simulink model "drive_esc"  (R2026b)
settings: Solver=VariableStepAuto
undefined symbols (not defined in the file or in its folder): DiscIntNeverNeededParam, P
libraries: simulink x14, mcbpccprotrelaylib x10, sl_discontinuities x2, mcbpccswwdtimerlib x1, slpidlib x1
settings Model: Creator=aomar  LastModifiedBy=aomar

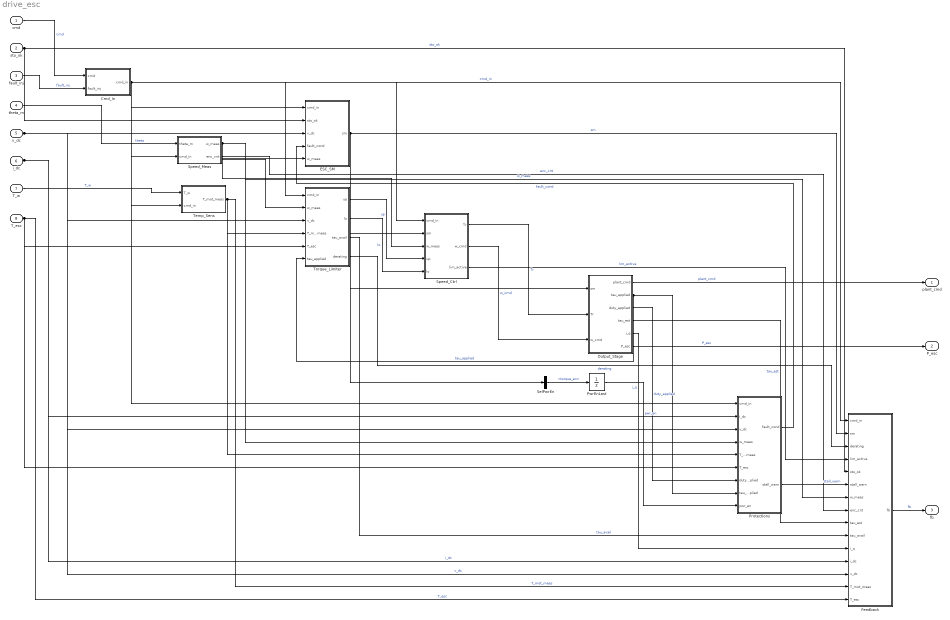
== system drive_esc ==
  cmd : Inport  OutDataTypeStr=Bus: Bus_DriveSideCmd  SampleTime=P.drive.Ts_esc
  sto_ok : Inport  Port=2  OutDataTypeStr=boolean  SampleTime=P.drive.Ts_esc
  fault_inj : Inport  Port=3  OutDataTypeStr=Bus: Bus_DriveSideFaultInj  SampleTime=P.drive.Ts_esc
  theta_m : Inport  Port=4  OutDataTypeStr=double  SampleTime=P.drive.Ts_esc
  v_dc : Inport  Port=5  OutDataTypeStr=double  SampleTime=P.drive.Ts_esc
  i_dc : Inport  Port=6  OutDataTypeStr=double  SampleTime=P.drive.Ts_esc
  T_w : Inport  Port=7  OutDataTypeStr=double  SampleTime=P.drive.Ts_esc
  T_esc : Inport  Port=8  OutDataTypeStr=double  SampleTime=P.drive.Ts_esc
  Cmd_In : Subsystem
  ESC_SM : Subsystem
  Feedback : Subsystem
  Output_Stage : Subsystem
  Protections : Subsystem
  PwrEnLast : UnitDelay  InitialCondition=false  SampleTime=P.drive.Ts_esc
  SelPwrEn : BusSelector  OutputSignals=torque_en
  Speed_Ctrl : Subsystem
  Speed_Meas : Subsystem
  Temp_Sens : Subsystem
  Torque_Limiter : Subsystem
  plant_cmd : Outport  OutDataTypeStr=double
  P_esc : Outport  Port=2  OutDataTypeStr=double
  fb : Outport  Port=3  OutDataTypeStr=Bus: Bus_DriveSideFb
  wires:
  cmd/1 -> Cmd_In/1(cmd)  "cmd"
  sto_ok/1 -> Feedback/5(sto_ok), ESC_SM/2(sto_ok)  "sto_ok"
  fault_inj/1 -> Cmd_In/2(fault_inj)  "fault_inj"
  theta_m/1 -> Speed_Meas/1(theta_m)  "theta"
  T_w/1 -> Temp_Sens/1(T_w)  "T_w"
  Cmd_In/1(cmd_in) -> Feedback/1(cmd_in), Protections/1(cmd_in), Speed_Ctrl/1(cmd_in), Temp_Sens/2(cmd_in), Torque_Limiter/1(cmd_in), Speed_Meas/2(cmd_in), ESC_SM/1(cmd_in)  "cmd_in"
  Speed_Meas/1(w_meas) -> Feedback/7(w_meas), Protections/4(w_meas), Speed_Ctrl/3(w_meas), Torque_Limiter/2(w_meas), ESC_SM/5(w_meas)  "w_meas"
  Speed_Meas/2(enc_cnt) -> Feedback/8(enc_cnt)  "enc_cnt"
  Temp_Sens/1(T_mot_meas) -> Feedback/14(T_mot_meas), Protections/5(T_mot_meas), Torque_Limiter/4(T_mot_meas)  "T_mot_meas"
  ESC_SM/1(sm) -> Feedback/2(sm), SelPwrEn/1, Output_Stage/1(sm), Speed_Ctrl/2(sm)  "sm"
  Torque_Limiter/1(up) -> Speed_Ctrl/4(up)  "up"
  Torque_Limiter/2(lo) -> Speed_Ctrl/5(lo)  "lo"
  Torque_Limiter/3(tau_avail) -> Feedback/10(tau_avail)  "tau_avail"
  Torque_Limiter/4(derating) -> Feedback/3(derating)  "derating"
  Speed_Ctrl/1(Tr) -> Output_Stage/2(Tr)  "Tr"
  Speed_Ctrl/2(w_cmd) -> Output_Stage/3(w_cmd)  "w_cmd"
  Speed_Ctrl/3(lim_active) -> Feedback/4(lim_active)  "lim_active"
  SelPwrEn/1 -> PwrEnLast/1  "<torque_en>"
  PwrEnLast/1 -> Protections/9(pwr_en)  "pwr_en"
  Output_Stage/1(plant_cmd) -> plant_cmd/1  "plant_cmd"
  Output_Stage/2(tau_applied) -> Protections/8(tau_applied), Torque_Limiter/6(tau_applied)  "tau_applied"
  Output_Stage/3(duty_applied) -> Protections/7(duty_applied)  "duty_applied"
  Output_Stage/4(tau_est) -> Feedback/9(tau_est)  "tau_est"
  Output_Stage/5(i_q) -> Feedback/11(i_q)  "i_q"
  Output_Stage/6(P_esc) -> P_esc/1  "P_esc"
  Protections/1(fault_cond) -> ESC_SM/4(fault_cond)  "fault_cond"
  Protections/2(stall_warn) -> Feedback/6(stall_warn)  "stall_warn"
  Feedback/1(fb) -> fb/1  "fb"
  v_dc/1 -> Feedback/13(v_dc), Protections/3(v_dc), Torque_Limiter/3(v_dc), ESC_SM/3(v_dc)  "v_dc"
  i_dc/1 -> Feedback/12(i_dc), Protections/2(i_dc)  "i_dc"
  T_esc/1 -> Feedback/15(T_esc), Protections/6(T_esc), Torque_Limiter/5(T_esc)  "T_esc"

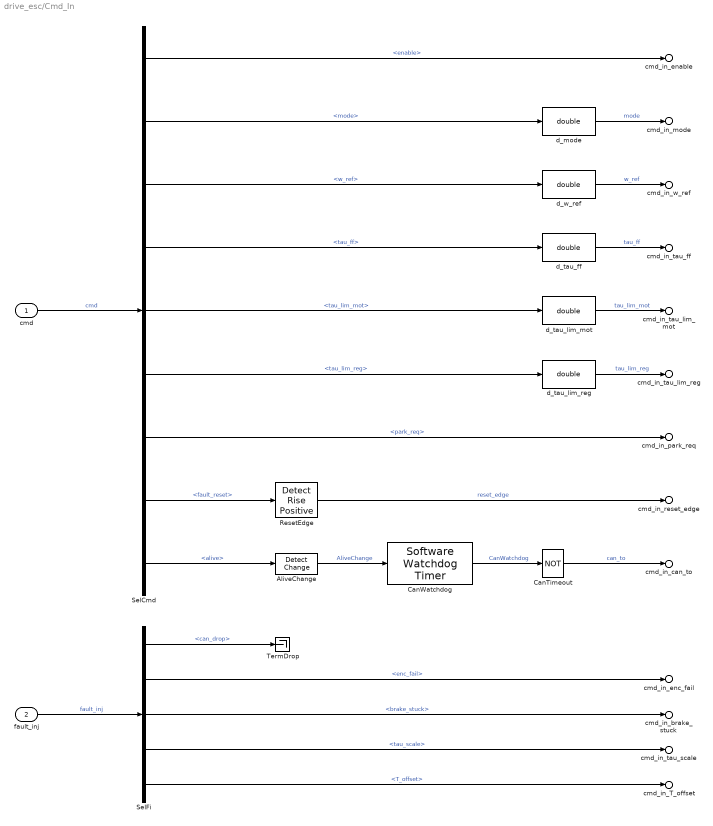
== system drive_esc/Cmd_In ==
  cmd : Inport
  fault_inj : Inport  Port=2
  AliveChange : simulink/Logic and Bit Operations/Detect Change  vinit=0  OutDataTypeStr=boolean
  CanTimeout : Logic  Operator=NOT  Inputs=1  AllPortsSameDT=off  OutDataTypeStr=boolean
  CanWatchdog : mcbpccswwdtimerlib/Software Watchdog Timer  maxCountInput=Specify via dialog  maxCount=P.drive.esc.n_can_to  datatype=uint8
      settings: LibrarySourceBlock=mcblib/Protection and Diagnostics/Software Watchdog Timer
  ResetEdge : simulink/Logic and Bit Operations/Detect Rise Positive  vinit=0  OutDataTypeStr=boolean
  SelCmd : BusSelector  OutputSignals=enable,mode,w_ref,tau_ff,tau_lim_mot,tau_lim_reg,park_req,fault_reset,alive
  SelFi : BusSelector  OutputSignals=can_drop,enc_fail,brake_stuck,tau_scale,T_offset
  TermDrop : Terminator
  d_mode : DataTypeConversion  OutDataTypeStr=double  RndMeth=Nearest
  d_tau_ff : DataTypeConversion  OutDataTypeStr=double  RndMeth=Nearest
  d_tau_lim_mot : DataTypeConversion  OutDataTypeStr=double  RndMeth=Nearest
  d_tau_lim_reg : DataTypeConversion  OutDataTypeStr=double  RndMeth=Nearest
  d_w_ref : DataTypeConversion  OutDataTypeStr=double  RndMeth=Nearest
  cmd_in_enable : Outport  PortName=cmd_in  Element=enable
  cmd_in_mode : Outport  PortName=cmd_in  Element=mode
  cmd_in_w_ref : Outport  PortName=cmd_in  Element=w_ref
  cmd_in_tau_ff : Outport  PortName=cmd_in  Element=tau_ff
  cmd_in_tau_lim_mot : Outport  PortName=cmd_in  Element=tau_lim_mot
  cmd_in_tau_lim_reg : Outport  PortName=cmd_in  Element=tau_lim_reg
  cmd_in_park_req : Outport  PortName=cmd_in  Element=park_req
  cmd_in_reset_edge : Outport  PortName=cmd_in  Element=reset_edge
  cmd_in_can_to : Outport  PortName=cmd_in  Element=can_to
  cmd_in_enc_fail : Outport  PortName=cmd_in  Element=enc_fail
  cmd_in_brake_stuck : Outport  PortName=cmd_in  Element=brake_stuck
  cmd_in_tau_scale : Outport  PortName=cmd_in  Element=tau_scale
  cmd_in_T_offset : Outport  PortName=cmd_in  Element=T_offset
  wires:
  cmd/1 -> SelCmd/1  "cmd"
  fault_inj/1 -> SelFi/1  "fault_inj"
  SelCmd/1 -> cmd_in_enable/1  "<enable>"
  SelCmd/2 -> d_mode/1  "<mode>"
  SelCmd/3 -> d_w_ref/1  "<w_ref>"
  SelCmd/4 -> d_tau_ff/1  "<tau_ff>"
  SelCmd/5 -> d_tau_lim_mot/1  "<tau_lim_mot>"
  SelCmd/6 -> d_tau_lim_reg/1  "<tau_lim_reg>"
  SelCmd/7 -> cmd_in_park_req/1  "<park_req>"
  SelCmd/8 -> ResetEdge/1  "<fault_reset>"
  SelCmd/9 -> AliveChange/1  "<alive>"
  SelFi/1 -> TermDrop/1  "<can_drop>"
  SelFi/2 -> cmd_in_enc_fail/1  "<enc_fail>"
  SelFi/3 -> cmd_in_brake_stuck/1  "<brake_stuck>"
  SelFi/4 -> cmd_in_tau_scale/1  "<tau_scale>"
  SelFi/5 -> cmd_in_T_offset/1  "<T_offset>"
  ResetEdge/1 -> cmd_in_reset_edge/1  "reset_edge"
  AliveChange/1 -> CanWatchdog/1  "AliveChange"
  CanWatchdog/1 -> CanTimeout/1  "CanWatchdog"
  CanTimeout/1 -> cmd_in_can_to/1  "can_to"
  d_mode/1 -> cmd_in_mode/1  "mode"
  d_w_ref/1 -> cmd_in_w_ref/1  "w_ref"
  d_tau_ff/1 -> cmd_in_tau_ff/1  "tau_ff"
  d_tau_lim_mot/1 -> cmd_in_tau_lim_mot/1  "tau_lim_mot"
  d_tau_lim_reg/1 -> cmd_in_tau_lim_reg/1  "tau_lim_reg"

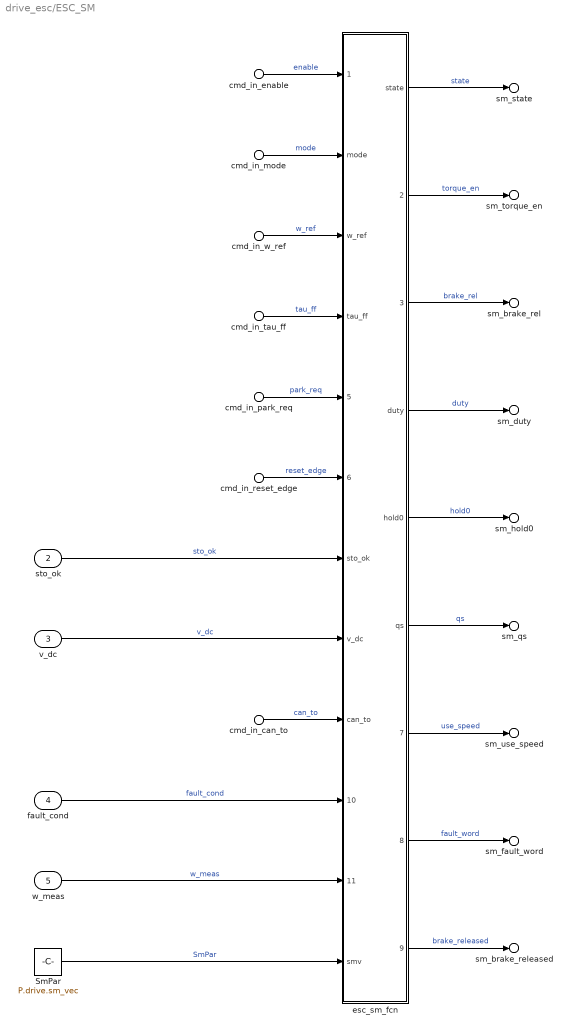
== system drive_esc/ESC_SM ==
  cmd_in_enable : Inport  PortName=cmd_in  Element=enable
  cmd_in_mode : Inport  PortName=cmd_in  Element=mode
  cmd_in_w_ref : Inport  PortName=cmd_in  Element=w_ref
  cmd_in_tau_ff : Inport  PortName=cmd_in  Element=tau_ff
  cmd_in_park_req : Inport  PortName=cmd_in  Element=park_req
  cmd_in_reset_edge : Inport  PortName=cmd_in  Element=reset_edge
  cmd_in_can_to : Inport  PortName=cmd_in  Element=can_to
  sto_ok : Inport  Port=2
  v_dc : Inport  Port=3
  fault_cond : Inport  Port=4
  w_meas : Inport  Port=5
  SmPar : Constant  Value=P.drive.sm_vec  OutDataTypeStr=double
  esc_sm_fcn : MATLAB Function  TreatAsAtomicUnit=on
  sm_state : Outport  PortName=sm  Element=state
  sm_torque_en : Outport  PortName=sm  Element=torque_en
  sm_brake_rel : Outport  PortName=sm  Element=brake_rel
  sm_duty : Outport  PortName=sm  Element=duty
  sm_hold0 : Outport  PortName=sm  Element=hold0
  sm_qs : Outport  PortName=sm  Element=qs
  sm_use_speed : Outport  PortName=sm  Element=use_speed
  sm_fault_word : Outport  PortName=sm  Element=fault_word
  sm_brake_released : Outport  PortName=sm  Element=brake_released
  wires:
  sto_ok/1 -> esc_sm_fcn/7(sto_ok)  "sto_ok"
  v_dc/1 -> esc_sm_fcn/8(v_dc)  "v_dc"
  fault_cond/1 -> esc_sm_fcn/10(fault_cond)  "fault_cond"
  w_meas/1 -> esc_sm_fcn/11(w_meas)  "w_meas"
  SmPar/1 -> esc_sm_fcn/12(smv)  "SmPar"
  cmd_in_enable/1 -> esc_sm_fcn/1(enable)  "enable"
  cmd_in_mode/1 -> esc_sm_fcn/2(mode)  "mode"
  cmd_in_w_ref/1 -> esc_sm_fcn/3(w_ref)  "w_ref"
  cmd_in_tau_ff/1 -> esc_sm_fcn/4(tau_ff)  "tau_ff"
  cmd_in_park_req/1 -> esc_sm_fcn/5(park_req)  "park_req"
  cmd_in_reset_edge/1 -> esc_sm_fcn/6(reset_edge)  "reset_edge"
  cmd_in_can_to/1 -> esc_sm_fcn/9(can_to)  "can_to"
  esc_sm_fcn/1(state) -> sm_state/1  "state"
  esc_sm_fcn/2(torque_en) -> sm_torque_en/1  "torque_en"
  esc_sm_fcn/3(brake_rel) -> sm_brake_rel/1  "brake_rel"
  esc_sm_fcn/4(duty) -> sm_duty/1  "duty"
  esc_sm_fcn/5(hold0) -> sm_hold0/1  "hold0"
  esc_sm_fcn/6(qs) -> sm_qs/1  "qs"
  esc_sm_fcn/7(use_speed) -> sm_use_speed/1  "use_speed"
  esc_sm_fcn/8(fault_word) -> sm_fault_word/1  "fault_word"
  esc_sm_fcn/9(brake_released) -> sm_brake_released/1  "brake_released"

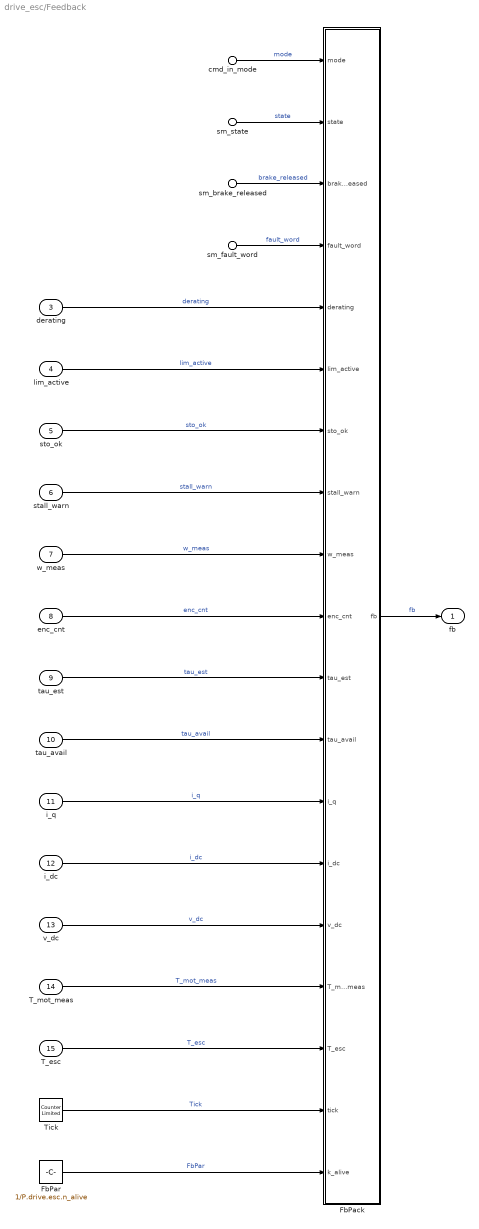
== system drive_esc/Feedback ==
  cmd_in_mode : Inport  PortName=cmd_in  Element=mode
  sm_state : Inport  Port=2  PortName=sm  Element=state
  sm_brake_released : Inport  Port=2  PortName=sm  Element=brake_released
  sm_fault_word : Inport  Port=2  PortName=sm  Element=fault_word
  derating : Inport  Port=3
  lim_active : Inport  Port=4
  sto_ok : Inport  Port=5
  stall_warn : Inport  Port=6
  w_meas : Inport  Port=7
  enc_cnt : Inport  Port=8
  tau_est : Inport  Port=9
  tau_avail : Inport  Port=10
  i_q : Inport  Port=11
  i_dc : Inport  Port=12
  v_dc : Inport  Port=13
  T_mot_meas : Inport  Port=14
  T_esc : Inport  Port=15
  FbPack : MATLAB Function  TreatAsAtomicUnit=on
  FbPar : Constant  Value=1/P.drive.esc.n_alive  OutDataTypeStr=double
  Tick : simulink/Sources/Counter Limited  uplimit=256*P.drive.esc.n_alive - 1  tsamp=P.drive.Ts_esc
  fb : Outport
  wires:
  derating/1 -> FbPack/5(derating)  "derating"
  lim_active/1 -> FbPack/6(lim_active)  "lim_active"
  sto_ok/1 -> FbPack/7(sto_ok)  "sto_ok"
  stall_warn/1 -> FbPack/8(stall_warn)  "stall_warn"
  w_meas/1 -> FbPack/9(w_meas)  "w_meas"
  enc_cnt/1 -> FbPack/10(enc_cnt)  "enc_cnt"
  tau_est/1 -> FbPack/11(tau_est)  "tau_est"
  tau_avail/1 -> FbPack/12(tau_avail)  "tau_avail"
  i_q/1 -> FbPack/13(i_q)  "i_q"
  i_dc/1 -> FbPack/14(i_dc)  "i_dc"
  v_dc/1 -> FbPack/15(v_dc)  "v_dc"
  T_mot_meas/1 -> FbPack/16(T_mot_meas)  "T_mot_meas"
  T_esc/1 -> FbPack/17(T_esc)  "T_esc"
  Tick/1 -> FbPack/18(tick)  "Tick"
  FbPar/1 -> FbPack/19(k_alive)  "FbPar"
  cmd_in_mode/1 -> FbPack/1(mode)  "mode"
  sm_state/1 -> FbPack/2(state)  "state"
  sm_brake_released/1 -> FbPack/3(brake_released)  "brake_released"
  sm_fault_word/1 -> FbPack/4(fault_word)  "fault_word"
  FbPack/1(fb) -> fb/1  "fb"

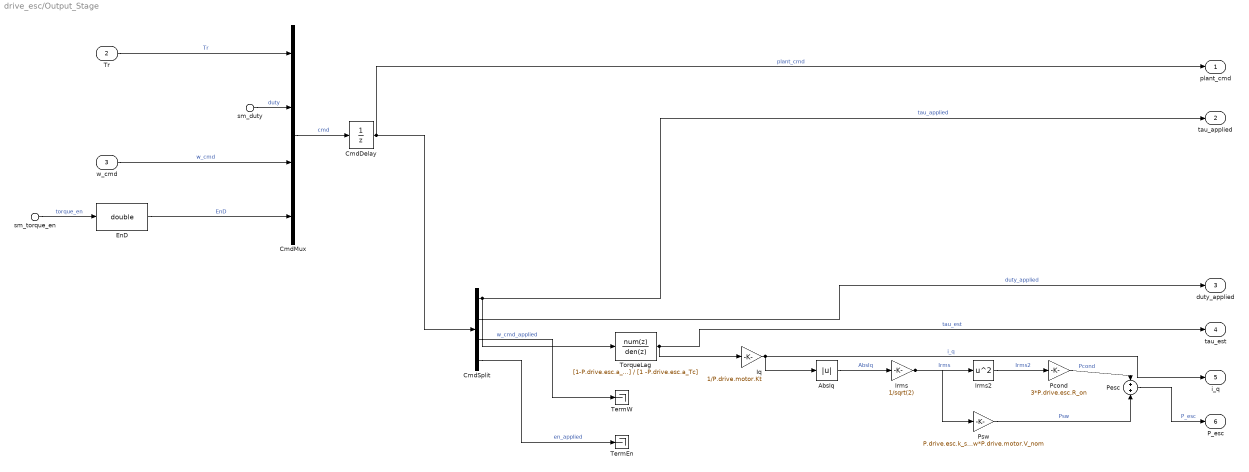
== system drive_esc/Output_Stage ==
  sm_duty : Inport  PortName=sm  Element=duty
  sm_torque_en : Inport  PortName=sm  Element=torque_en
  Tr : Inport  Port=2
  w_cmd : Inport  Port=3
  AbsIq : Abs  SaturateOnIntegerOverflow=off
  CmdDelay : UnitDelay  InitialCondition=zeros(4,1)  SampleTime=P.drive.Ts_esc
  CmdMux : Mux
  CmdSplit : Demux
  EnD : DataTypeConversion  OutDataTypeStr=double  RndMeth=Nearest
  Iq : Gain  Gain=1/P.drive.motor.Kt
  Irms : Gain  Gain=1/sqrt(2)
  Irms2 : Math  Operator=square
  Pcond : Gain  Gain=3*P.drive.esc.R_on
  Pesc : Sum
  Psw : Gain  Gain=P.drive.esc.k_sw*P.drive.motor.V_nom
  TermEn : Terminator
  TermW : Terminator
  TorqueLag : DiscreteTransferFcn  Numerator=[1-P.drive.esc.a_Tc]  Denominator=[1 -P.drive.esc.a_Tc]  SampleTime=P.drive.Ts_esc
  plant_cmd : Outport
  tau_applied : Outport  Port=2
  duty_applied : Outport  Port=3
  tau_est : Outport  Port=4
  i_q : Outport  Port=5
  P_esc : Outport  Port=6
  wires:
  sm_torque_en/1 -> EnD/1  "torque_en"
  Tr/1 -> CmdMux/1  "Tr"
  w_cmd/1 -> CmdMux/3  "w_cmd"
  EnD/1 -> CmdMux/4  "EnD"
  sm_duty/1 -> CmdMux/2  "duty"
  CmdMux/1 -> CmdDelay/1  "cmd"
  CmdDelay/1 -> CmdSplit/1, plant_cmd/1  "plant_cmd"
  CmdSplit/1 -> tau_applied/1, TorqueLag/1  "tau_applied"
  CmdSplit/2 -> duty_applied/1  "duty_applied"
  CmdSplit/3 -> TermW/1  "w_cmd_applied"
  CmdSplit/4 -> TermEn/1  "en_applied"
  TorqueLag/1 -> tau_est/1, Iq/1  "tau_est"
  Iq/1 -> i_q/1, AbsIq/1  "i_q"
  AbsIq/1 -> Irms/1  "AbsIq"
  Irms/1 -> Psw/1, Irms2/1  "Irms"
  Irms2/1 -> Pcond/1  "Irms2"
  Psw/1 -> Pesc/2  "Psw"
  Pcond/1 -> Pesc/1  "Pcond"
  Pesc/1 -> P_esc/1  "P_esc"

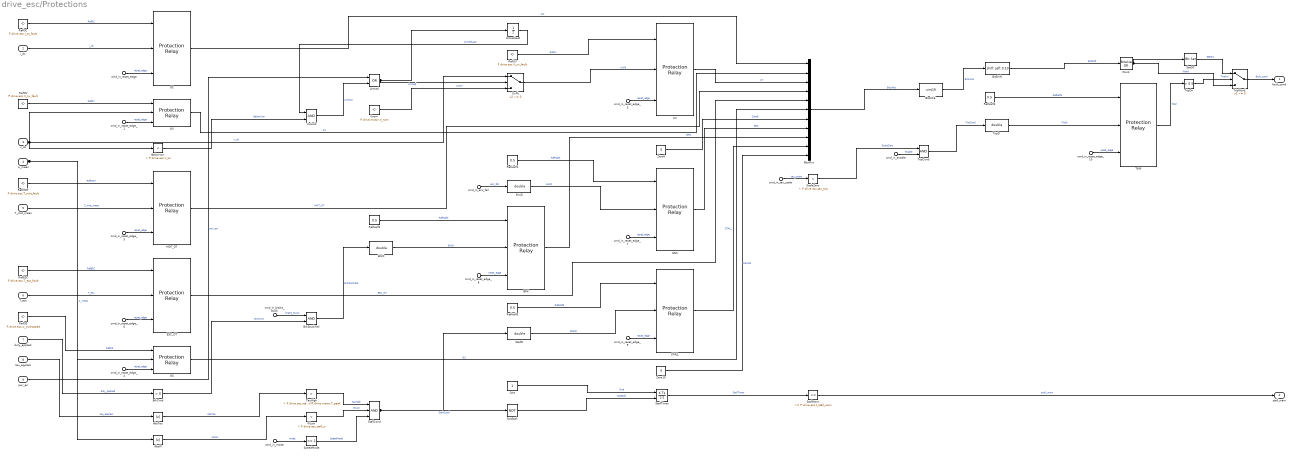
== system drive_esc/Protections ==
  cmd_in_enc_fail : Inport  PortName=cmd_in  Element=enc_fail
  cmd_in_brake_stuck : Inport  PortName=cmd_in  Element=brake_stuck
  cmd_in_mode : Inport  PortName=cmd_in  Element=mode
  cmd_in_tau_scale : Inport  PortName=cmd_in  Element=tau_scale
  cmd_in_enable : Inport  PortName=cmd_in  Element=enable
  cmd_in_reset_edge : Inport  PortName=cmd_in  Element=reset_edge
  cmd_in_reset_edge_{2..10} (9 alike) : Inport  PortName=cmd_in  Element=reset_edge
  i_dc : Inport  Port=2
  v_dc : Inport  Port=3
  w_meas : Inport  Port=4
  T_mot_meas : Inport  Port=5
  T_esc : Inport  Port=6
  duty_applied : Inport  Port=7
  tau_applied : Inport  Port=8
  pwr_en : Inport  Port=9
  AbsTau : Abs  SaturateOnIntegerOverflow=off
  AbsW : Abs  SaturateOnIntegerOverflow=off
  Armed : Logic  Operator=OR  AllPortsSameDT=off  OutDataTypeStr=boolean
  ArmedLast : UnitDelay  InitialCondition=false  SampleTime=P.drive.Ts_esc
  BRK : mcbpccprotrelaylib/Protection Relay  Protection=Overvoltage  CountMaxInputType=Specify via dialog  CountMax=P.drive.esc.n_brake  SamplesForDebounce=0
      settings: LibrarySourceBlock=mcblib/Protection and Diagnostics/Protection Relay
  BelowVon : simulink/Logic and Bit Operations/Compare To Constant  relop=<  const=P.drive.esc.V_on  OutDataTypeStr=boolean
  BitShift : ArithShift  BitShiftNumber=0:10  BitShiftDirection=Left
  BitsMux : Mux  Inputs=11
  BitsU16 : DataTypeConversion  OutDataTypeStr=uint16  RndMeth=Nearest
  BrkCmd : simulink/Logic and Bit Operations/Compare To Constant  relop=>  const=0  OutDataTypeStr=boolean
  BrkD : DataTypeConversion  OutDataTypeStr=double  RndMeth=Nearest
  BrkStuckRel : Logic  AllPortsSameDT=off  OutDataTypeStr=boolean
  ENC : mcbpccprotrelaylib/Protection Relay  Protection=Overvoltage  CountMaxInputType=Specify via dialog  CountMax=P.drive.esc.n_enc  SamplesForDebounce=0
      settings: LibrarySourceBlock=mcblib/Protection and Diagnostics/Protection Relay
  ESC_OT : mcbpccprotrelaylib/Protection Relay  Protection=Overvoltage  CountMaxInputType=Specify via dialog  CountMax=P.drive.esc.n_ot  SamplesForDebounce=0
      settings: LibrarySourceBlock=mcblib/Protection and Diagnostics/Protection Relay
  EncD : DataTypeConversion  OutDataTypeStr=double  RndMeth=Nearest
  MOT_OT : mcbpccprotrelaylib/Protection Relay  Protection=Overvoltage  CountMaxInputType=Specify via dialog  CountMax=P.drive.esc.n_ot  SamplesForDebounce=0
      settings: LibrarySourceBlock=mcblib/Protection and Diagnostics/Protection Relay
  NotStall : Logic  Operator=NOT  Inputs=1  AllPortsSameDT=off  OutDataTypeStr=boolean
  OC : mcbpccprotrelaylib/Protection Relay  Protection=Overcurrent  CountMaxInputType=Specify via dialog  CountMax=P.drive.esc.n_oc  SamplesForDebounce=0
      settings: LibrarySourceBlock=mcblib/Protection and Diagnostics/Protection Relay
  OS : mcbpccprotrelaylib/Protection Relay  Protection=Overspeed  CountMaxInputType=Specify via dialog  CountMax=P.drive.esc.n_os  SamplesForDebounce=0
      settings: LibrarySourceBlock=mcblib/Protection and Diagnostics/Protection Relay
  OV : mcbpccprotrelaylib/Protection Relay  Protection=Overvoltage  CountMaxInputType=Specify via dialog  CountMax=P.drive.esc.n_ov  SamplesForDebounce=0
      settings: LibrarySourceBlock=mcblib/Protection and Diagnostics/Protection Relay
  One : Constant
  RefESC : Constant  Value=P.drive.esc.T_esc_fault
  RefHalf{1..4} (4 alike) : Constant  Value=0.5
  RefMOT : Constant  Value=P.drive.esc.T_mot_fault
  RefOC : Constant  Value=P.drive.esc.I_oc_fault
  RefOS : Constant  Value=P.drive.esc.w_overspeed
  RefOV : Constant  Value=P.drive.esc.V_ov_fault
  RefUV : Constant  Value=P.drive.esc.V_uv_fault
  STALL : mcbpccprotrelaylib/Protection Relay  Protection=Overvoltage  CountMaxInputType=Specify via dialog  CountMax=P.drive.esc.n_stall  SamplesForDebounce=0
      settings: LibrarySourceBlock=mcblib/Protection and Diagnostics/Protection Relay
  ScaleZero : simulink/Logic and Bit Operations/Compare To Constant  relop=<  const=P.drive.esc.tau_trip  OutDataTypeStr=boolean
  SetOC : simulink/Logic and Bit Operations/Bit Set  iBit=0
  SpeedMode : simulink/Logic and Bit Operations/Compare To Constant  relop===  const=1  OutDataTypeStr=boolean
  StallCond : Logic  Inputs=3  AllPortsSameDT=off  OutDataTypeStr=boolean
  StallD : DataTypeConversion  OutDataTypeStr=double  RndMeth=Nearest
  StallTimer : DiscreteIntegrator  ExternalReset=level  SampleTime=P.drive.Ts_esc  ICPrevOutput=DiscIntNeverNeededParam  ICPrevScaledInput=DiscIntNeverNeededParam
  StallWarn : simulink/Logic and Bit Operations/Compare To Constant  relop=>=  const=P.drive.esc.t_stall_warn  OutDataTypeStr=boolean
  TRIP : mcbpccprotrelaylib/Protection Relay  Protection=Overvoltage  CountMaxInputType=Specify via dialog  CountMax=1  SamplesForDebounce=0
      settings: LibrarySourceBlock=mcblib/Protection and Diagnostics/Protection Relay
  TauHigh : simulink/Logic and Bit Operations/Compare To Constant  relop=>  const=P.drive.esc.stall_tau_frac*P.drive.motor.T_peak  OutDataTypeStr=boolean
  TripCond : Logic  AllPortsSameDT=off  OutDataTypeStr=boolean
  TripD : DataTypeConversion  OutDataTypeStr=double  RndMeth=Nearest
  TripOn : simulink/Logic and Bit Operations/Compare To Constant  relop=>  const=0.5  OutDataTypeStr=boolean
  TripWord : Switch  Criteria=u2 ~= 0  SaturateOnIntegerOverflow=off  InputSameDT=off
  UV : mcbpccprotrelaylib/Protection Relay  Protection=Undervoltage  CountMaxInputType=Specify via dialog  CountMax=P.drive.esc.n_uv  SamplesForDebounce=0
      settings: LibrarySourceBlock=mcblib/Protection and Diagnostics/Protection Relay
  UvFb : Switch  Criteria=u2 ~= 0  SaturateOnIntegerOverflow=off  InputSameDT=off
  UvHold : Logic  AllPortsSameDT=off  OutDataTypeStr=boolean
  Vnom : Constant  Value=P.drive.motor.V_nom
  WLow : simulink/Logic and Bit Operations/Compare To Constant  relop=<  const=P.drive.esc.stall_w  OutDataTypeStr=boolean
  Word : simulink/Logic and Bit Operations/Bitwise Operator  logicop=OR  UseBitMask=off  BitMask=bin2dec('11011001')  BitMaskRealWorld=Stored Integer
  Zero10 : Constant  Value=0
  Zero6 : Constant  Value=0
  fault_cond : Outport
  stall_warn : Outport  Port=2
  wires:
  RefOC/1 -> OC/1  "RefOC"
  i_dc/1 -> OC/2  "i_dc"
  RefOV/1 -> OV/1  "RefOV"
  v_dc/1 -> UvFb/1, OV/2, BelowVon/1  "v_dc"
  w_meas/1 -> AbsW/1, OS/2  "w_meas"
  RefMOT/1 -> MOT_OT/1  "RefMOT"
  T_mot_meas/1 -> MOT_OT/2  "T_mot_meas"
  RefESC/1 -> ESC_OT/1  "RefESC"
  T_esc/1 -> ESC_OT/2  "T_esc"
  RefOS/1 -> OS/1  "RefOS"
  duty_applied/1 -> BrkCmd/1  "duty_applied"
  tau_applied/1 -> AbsTau/1  "tau_applied"
  pwr_en/1 -> Armed/1  "pwr_en"
  cmd_in_reset_edge/1 -> OC/3  "reset_edge"
  cmd_in_reset_edge_2/1 -> OV/3  "reset_edge"
  cmd_in_reset_edge_5/1 -> MOT_OT/3  "reset_edge"
  cmd_in_reset_edge_6/1 -> ESC_OT/3  "reset_edge"
  cmd_in_reset_edge_4/1 -> OS/3  "reset_edge"
  BelowVon/1 -> UvHold/2  "BelowVon"
  BrkCmd/1 -> BrkStuckRel/2  "BrkCmd"
  AbsTau/1 -> TauHigh/1  "AbsTau"
  AbsW/1 -> WLow/1  "AbsW"
  OC/1 -> BitsMux/1  "OC"
  OV/1 -> BitsMux/2  "OV"
  MOT_OT/1 -> BitsMux/4  "MOT_OT"
  ESC_OT/1 -> BitsMux/5  "ESC_OT"
  OS/1 -> BitsMux/6  "OS"
  cmd_in_brake_stuck/1 -> BrkStuckRel/1  "brake_stuck"
  cmd_in_mode/1 -> SpeedMode/1  "mode"
  UvHold/1 -> Armed/2  "UvHold"
  BrkStuckRel/1 -> BrkD/1  "BrkStuckRel"
  TauHigh/1 -> StallCond/1  "TauHigh"
  WLow/1 -> StallCond/2  "WLow"
  SpeedMode/1 -> StallCond/3  "SpeedMode"
  Armed/1 -> ArmedLast/1, UvFb/2  "Armed"
  Vnom/1 -> UvFb/3  "Vnom"
  RefHalf2/1 -> BRK/1  "RefHalf2"
  StallCond/1 -> StallD/1, NotStall/1  "StallCond"
  BrkD/1 -> BRK/2  "BrkD"
  cmd_in_enc_fail/1 -> EncD/1  "enc_fail"
  cmd_in_reset_edge_8/1 -> BRK/3  "reset_edge"
  RefUV/1 -> UV/1  "RefUV"
  RefHalf1/1 -> ENC/1  "RefHalf1"
  RefHalf3/1 -> STALL/1  "RefHalf3"
  One/1 -> StallTimer/1  "One"
  NotStall/1 -> StallTimer/2  "NotStall"
  ArmedLast/1 -> UvHold/1  "ArmedLast"
  UvFb/1 -> UV/2  "UvFb"
  EncD/1 -> ENC/2  "EncD"
  StallD/1 -> STALL/2  "StallD"
  BRK/1 -> BitsMux/9  "BRK"
  cmd_in_reset_edge_3/1 -> UV/3  "reset_edge"
  cmd_in_reset_edge_7/1 -> ENC/3  "reset_edge"
  cmd_in_reset_edge_9/1 -> STALL/3  "reset_edge"
  Zero6/1 -> BitsMux/7  "Zero6"
  Zero10/1 -> BitsMux/11  "Zero10"
  StallTimer/1 -> StallWarn/1  "StallTimer"
  UV/1 -> BitsMux/3  "UV"
  ENC/1 -> BitsMux/8  "ENC"
  STALL/1 -> BitsMux/10  "STALL"
  cmd_in_tau_scale/1 -> ScaleZero/1  "tau_scale"
  BitsMux/1 -> BitsU16/1  "BitsMux"
  ScaleZero/1 -> TripCond/1  "ScaleZero"
  StallWarn/1 -> stall_warn/1  "stall_warn"
  cmd_in_enable/1 -> TripCond/2  "enable"
  TripCond/1 -> TripD/1  "TripCond"
  BitsU16/1 -> BitShift/1  "BitsU16"
  RefHalf4/1 -> TRIP/1  "RefHalf4"
  TripD/1 -> TRIP/2  "TripD"
  BitShift/1 -> Word/1  "BitShift"
  cmd_in_reset_edge_10/1 -> TRIP/3  "reset_edge"
  Word/1 -> TripWord/3, SetOC/1  "Word"
  TRIP/1 -> TripOn/1  "TRIP"
  TripOn/1 -> TripWord/2  "TripOn"
  SetOC/1 -> TripWord/1  "SetOC"
  TripWord/1 -> fault_cond/1  "fault_cond"

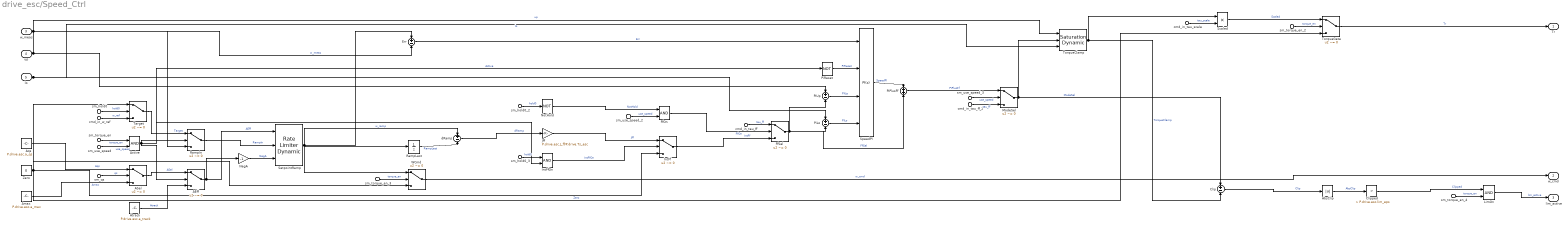
== system drive_esc/Speed_Ctrl ==
  cmd_in_w_ref : Inport  PortName=cmd_in  Element=w_ref
  cmd_in_tau_ff : Inport  PortName=cmd_in  Element=tau_ff
  cmd_in_tau_ff_2 : Inport  PortName=cmd_in  Element=tau_ff
  cmd_in_tau_scale : Inport  PortName=cmd_in  Element=tau_scale
  sm_hold0 : Inport  Port=2  PortName=sm  Element=hold0
  sm_hold0_2 : Inport  Port=2  PortName=sm  Element=hold0
  sm_hold0_3 : Inport  Port=2  PortName=sm  Element=hold0
  sm_torque_en : Inport  Port=2  PortName=sm  Element=torque_en
  sm_torque_en_2 : Inport  Port=2  PortName=sm  Element=torque_en
  sm_torque_en_3 : Inport  Port=2  PortName=sm  Element=torque_en
  sm_torque_en_4 : Inport  Port=2  PortName=sm  Element=torque_en
  sm_use_speed : Inport  Port=2  PortName=sm  Element=use_speed
  sm_use_speed_2 : Inport  Port=2  PortName=sm  Element=use_speed
  sm_use_speed_3 : Inport  Port=2  PortName=sm  Element=use_speed
  sm_qs : Inport  Port=2  PortName=sm  Element=qs
  w_meas : Inport  Port=3
  up : Inport  Port=4
  lo : Inport  Port=5
  AEff : Switch  Criteria=u2 ~= 0  SaturateOnIntegerOverflow=off  InputSameDT=off
  ASel : Switch  Criteria=u2 ~= 0  SaturateOnIntegerOverflow=off  InputSameDT=off
  AbsClip : Abs  SaturateOnIntegerOverflow=off
  Active : Logic  AllPortsSameDT=off  OutDataTypeStr=boolean
  Amax : Constant  Value=P.drive.esc.a_max
  Aqs : Constant  Value=P.drive.esc.a_qs
  Atrack : Constant  Value=P.drive.esc.a_track
  Clip : Sum  Inputs=+-
  Clipped : simulink/Logic and Bit Operations/Compare To Constant  relop=>  const=P.drive.esc.lim_eps  OutDataTypeStr=boolean
  Err : Sum  Inputs=+-
  FfOn : Logic  AllPortsSameDT=off  OutDataTypeStr=boolean
  FfSel : Switch  Criteria=u2 ~= 0  SaturateOnIntegerOverflow=off  InputSameDT=off
  IntFf : Switch  Criteria=u2 ~= 0  SaturateOnIntegerOverflow=off  InputSameDT=off
  IntFfOn : Logic  AllPortsSameDT=off  OutDataTypeStr=boolean
  Jff : Gain  Gain=P.drive.esc.J_ff/P.drive.Ts_esc
  LimOn : Logic  AllPortsSameDT=off  OutDataTypeStr=boolean
  ModeSel : Switch  Criteria=u2 ~= 0  SaturateOnIntegerOverflow=off  InputSameDT=off
  NegA : Gain  Gain=-1
  NotHold : Logic  Operator=NOT  Inputs=1  AllPortsSameDT=off  OutDataTypeStr=boolean
  PiLo : Sum  Inputs=+-
  PiPlusFf : Sum
  PiReset : Logic  Operator=NOT  Inputs=1  AllPortsSameDT=off  OutDataTypeStr=boolean
  PiUp : Sum  Inputs=+-
  RampIn : Switch  Criteria=u2 ~= 0  SaturateOnIntegerOverflow=off  InputSameDT=off
  RampLast : UnitDelay  SampleTime=P.drive.Ts_esc
  Scaled : Product  Inputs=**
  SetpointRamp : sl_discontinuities/Rate Limiter Dynamic
      settings: LibrarySourceBlock=|
      | simulink/Discontinuities/Rate Limiter
      | Dynamic
  SpeedPI : slpidlib/PID Controller  Controller=PI  Form=Parallel  TimeDomain=Discrete-time  UseExternalTs=off  SampleTime=P.drive.Ts_esc  IntegratorMethod=Backward Euler  FilterMethod=Forward Euler  ControllerParametersSource=internal  P=P.drive.esc.Kp_w  I=P.drive.esc.Ki_w  UseKiTs=off  D=0  UseExternalDerivativeSource=off  N=100  UseFilter=on  TunerSelectOption=Transfer Function Based (PID Tuner App)  InitialConditionSource=internal  InitialConditionForIntegrator=0  InitialConditionForFilter=0  DifferentiatorICPrevScaledInput=0  ExternalReset=level  TrackingMode=off  Kt=1  LimitOutput=on  SatLimitsSource=external  UpperSaturationLimit=inf  LowerSaturationLimit=-inf  LinearizeAsGain=off  AntiWindupMode=clamping  Kb=1  LimitIntegrator=off  UpperIntegratorSaturationLimit=inf  LowerIntegratorSaturationLimit=-inf  POutMin=[]  POutMax=[]  IOutMin=[]  IOutMax=[]  DOutMin=[]  DOutMax=[]  NOutMin=[]  NOutMax=[]  SumOutMin=[]  SumOutMax=[]  SaturationOutMin=[]  SaturationOutMax=[]  PParamMin=[]  PParamMax=[]  IParamMin=[]  IParamMax=[]  DParamMin=[]  DParamMax=[]  NParamMin=[]  NParamMax=[]  KbParamMin=[]  KbParamMax=[]  KtParamMin=[]  KtParamMax=[]  KbOutMin=[]  KbOutMax=[]  KtOutMin=[]  KtOutMax=[]  IntegratorOutMin=[]  IntegratorOutMax=[]  FilterOutMin=[]  FilterOutMax=[]  SumI1OutMin=[]  SumI1OutMax=[]  SumI2OutMin=[]  SumI2OutMax=[]  SumI3OutMin=[]  SumI3OutMax=[]  SumI4OutMin=[]  SumI4OutMax=[]  SumDOutMin=[]  SumDOutMax=[]  DifferentiatorOutMin=[]  DifferentiatorOutMax=[]  FilterDiffOutCoefMin=[]  FilterDiffOutCoefMax=[]  ReciprocalOutMin=[]  ReciprocalOutMax=[]  SumDenOutMin=[]  SumDenOutMax=[]  SumNumOutMin=[]  SumNumOutMax=[]  DivideOutMin=[]  DivideOutMax=[]  UdiffTsProdOutMin=[]  UdiffTsProdOutMax=[]  NTsProdOutMin=[]  NTsProdOutMax=[]  UintegralTsProdOutMin=[]  UintegralTsProdOutMax=[]  UngainTsProdOutMin=[]  UngainTsProdOutMax=[]  ClampingZeroOutDataTypeStr=Inherit: Inherit via back propagation  ClampingZeroOutMin=[]  ClampingZeroOutMax=[]  FilterDenConstantOutDataTypeStr=Inherit: Inherit via back propagation  FilterDenConstantOutMin=[]  FilterDenConstantOutMax=[]  PCopyOutDataTypeStr=Inherit: Inherit via back propagation  PCopyOutMin=[]  PCopyOutMax=[]  NCopyOutDataTypeStr=Inherit: Inherit via back propagation  NCopyOutMin=[]  NCopyOutMax=[]  IntegratorContinuousStateAttributes=''  IntegratorStateMustResolveToSignalObject=off  IntegratorRTWStateStorageClass=Auto  FilterContinuousStateAttributes=''  FilterStateMustResolveToSignalObject=off  FilterRTWStateStorageClass=Auto  ParallelPVariant=InternalParameters  IdealPVariant=Disabled  IVariant=InternalParameters  DVariant=Disabled  IntegratorVariant=Discrete  SatVariant=External  AWVariant=DiscClampingParallel  PCopyVariant=Disabled  TRVariant=Disabled  FdbkBlocksVariant=Feedback  IdealPFdbkVariant=Passthrough  SatFdbkVariant=Passthrough  DerivativeFilterVariant=Disabled  NVariant=Disabled  NCopyVariant=Disabled_SignalSpec  FilterICVariant=Disabled  IntegratorICVariant=InternalICs  ExternalResetVariant=ExternalReset  TRSumVariant=Passthrough  SumFdbkVariant=Enabled  SumVariant=Sum_PI  TsampFilterVariant=InternalTs  TsampNgainVariant=Passthrough  TsampIntegralVariant=Disabled_SignalSpec  ExternalSaturationOutDataTypeStr=Inherit: Same as second input  DerivativeSourceVariant=Disabled  PreIntVariant=InternalPreInt
      settings: LibrarySourceBlock=simulink/Discrete/Discrete PID Controller
  Target : Switch  Criteria=u2 ~= 0  SaturateOnIntegerOverflow=off  InputSameDT=off
  TorqueClamp : sl_discontinuities/Saturation Dynamic  OutMin=[]  OutMax=[]  OutDataTypeStr=Inherit: Same as second input  OutDataType=fixdt(1, 16)  OutScaling=2^-10  DoSatur=off
      settings: LibrarySourceBlock=|
      | simulink/Discontinuities/Saturation
      | Dynamic
  TorqueGate : Switch  Criteria=u2 ~= 0  SaturateOnIntegerOverflow=off  InputSameDT=off
  WCmd : Switch  Criteria=u2 ~= 0  SaturateOnIntegerOverflow=off  InputSameDT=off
  Zero : Constant  Value=0
  dRamp : Sum  Inputs=+-
  Tr : Outport
  w_cmd : Outport  Port=2
  lim_active : Outport  Port=3
  wires:
  w_meas/1 -> RampIn/3, Err/2  "w_meas"
  up/1 -> PiUp/1, TorqueClamp/1  "up"
  Aqs/1 -> ASel/1  "Aqs"
  sm_hold0/1 -> Target/2  "hold0"
  cmd_in_w_ref/1 -> Target/3  "w_ref"
  sm_torque_en/1 -> Active/1  "torque_en"
  sm_use_speed/1 -> Active/2  "use_speed"
  sm_qs/1 -> ASel/2  "qs"
  Active/1 -> PiReset/1, AEff/2, IntFfOn/2, RampIn/2  "Active"
  Atrack/1 -> AEff/3  "Atrack"
  Target/1 -> RampIn/1  "Target"
  ASel/1 -> AEff/1  "ASel"
  RampIn/1 -> SetpointRamp/2  "RampIn"
  AEff/1 -> SetpointRamp/1, NegA/1  "AEff"
  NegA/1 -> SetpointRamp/3  "NegA"
  SetpointRamp/1 -> Err/1, WCmd/1, dRamp/1, RampLast/1  "w_ramp"
  sm_torque_en_3/1 -> WCmd/2  "torque_en"
  Err/1 -> SpeedPI/1  "Err"
  RampLast/1 -> dRamp/2  "RampLast"
  WCmd/1 -> w_cmd/1  "w_cmd"
  dRamp/1 -> Jff/1  "dRamp"
  sm_hold0_2/1 -> NotHold/1  "hold0"
  sm_hold0_3/1 -> IntFfOn/1  "hold0"
  NotHold/1 -> FfOn/1  "NotHold"
  Jff/1 -> IntFf/1  "Jff"
  IntFfOn/1 -> IntFf/2  "IntFfOn"
  sm_use_speed_2/1 -> FfOn/2  "use_speed"
  FfOn/1 -> FfSel/2  "FfOn"
  IntFf/1 -> FfSel/3  "IntFf"
  cmd_in_tau_ff/1 -> FfSel/1  "tau_ff"
  FfSel/1 -> PiPlusFf/2, PiUp/2, PiLo/2  "FfSel"
  PiUp/1 -> SpeedPI/3  "PiUp"
  PiLo/1 -> SpeedPI/4  "PiLo"
  PiReset/1 -> SpeedPI/2  "PiReset"
  SpeedPI/1 -> PiPlusFf/1  "SpeedPI"
  PiPlusFf/1 -> ModeSel/1  "PiPlusFf"
  sm_use_speed_3/1 -> ModeSel/2  "use_speed"
  cmd_in_tau_ff_2/1 -> ModeSel/3  "tau_ff"
  ModeSel/1 -> Clip/1, TorqueClamp/2  "ModeSel"
  TorqueClamp/1 -> Clip/2, Scaled/1  "TorqueClamp"
  cmd_in_tau_scale/1 -> Scaled/2  "tau_scale"
  Clip/1 -> AbsClip/1  "Clip"
  Scaled/1 -> TorqueGate/1  "Scaled"
  sm_torque_en_2/1 -> TorqueGate/2  "torque_en"
  AbsClip/1 -> Clipped/1  "AbsClip"
  TorqueGate/1 -> Tr/1  "Tr"
  Clipped/1 -> LimOn/1  "Clipped"
  sm_torque_en_4/1 -> LimOn/2  "torque_en"
  LimOn/1 -> lim_active/1  "lim_active"
  Zero/1 -> IntFf/3, TorqueGate/3, Target/1, WCmd/3  "Zero"
  Amax/1 -> ASel/3  "Amax"
  lo/1 -> PiLo/1, TorqueClamp/3  "lo"

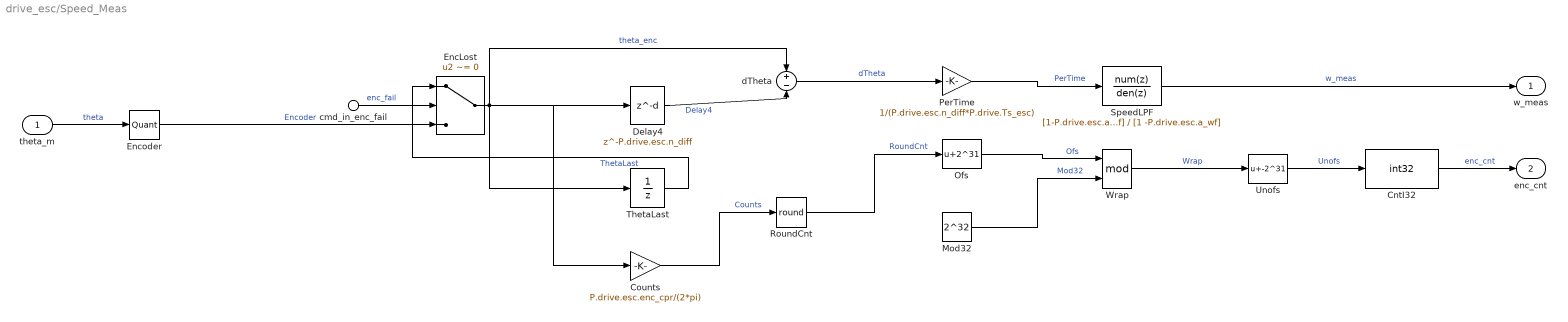
== system drive_esc/Speed_Meas ==
  theta_m : Inport
  cmd_in_enc_fail : Inport  Port=2  PortName=cmd_in  Element=enc_fail
  CntI32 : DataTypeConversion  OutDataTypeStr=int32  RndMeth=Nearest
  Counts : Gain  Gain=P.drive.esc.enc_cpr/(2*pi)
  Delay4 : Delay  DelayLength=P.drive.esc.n_diff  InitialCondition=0  SampleTime=P.drive.Ts_esc
  EncLost : Switch  Criteria=u2 ~= 0  SaturateOnIntegerOverflow=off  InputSameDT=off
  Encoder : Quantizer  QuantizationInterval=2*pi/P.drive.esc.enc_cpr  SampleTime=P.drive.Ts_esc
  Mod32 : Constant  Value=2^32
  Ofs : Bias  Bias=2^31  SaturateOnIntegerOverflow=off
  PerTime : Gain  Gain=1/(P.drive.esc.n_diff*P.drive.Ts_esc)
  RoundCnt : Rounding  Operator=round
  SpeedLPF : DiscreteTransferFcn  Numerator=[1-P.drive.esc.a_wf]  Denominator=[1 -P.drive.esc.a_wf]  SampleTime=P.drive.Ts_esc
  ThetaLast : UnitDelay  SampleTime=P.drive.Ts_esc
  Unofs : Bias  Bias=-2^31  SaturateOnIntegerOverflow=off
  Wrap : Math  Operator=mod
  dTheta : Sum  Inputs=+-
  w_meas : Outport
  enc_cnt : Outport  Port=2
  wires:
  theta_m/1 -> Encoder/1  "theta"
  Encoder/1 -> EncLost/3  "Encoder"
  cmd_in_enc_fail/1 -> EncLost/2  "enc_fail"
  EncLost/1 -> Counts/1, ThetaLast/1, dTheta/1, Delay4/1  "theta_enc"
  Counts/1 -> RoundCnt/1  "Counts"
  Delay4/1 -> dTheta/2  "Delay4"
  ThetaLast/1 -> EncLost/1  "ThetaLast"
  dTheta/1 -> PerTime/1  "dTheta"
  RoundCnt/1 -> Ofs/1  "RoundCnt"
  PerTime/1 -> SpeedLPF/1  "PerTime"
  Mod32/1 -> Wrap/2  "Mod32"
  Ofs/1 -> Wrap/1  "Ofs"
  Wrap/1 -> Unofs/1  "Wrap"
  SpeedLPF/1 -> w_meas/1  "w_meas"
  Unofs/1 -> CntI32/1  "Unofs"
  CntI32/1 -> enc_cnt/1  "enc_cnt"

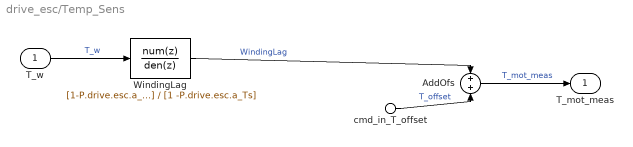
== system drive_esc/Temp_Sens ==
  T_w : Inport
  cmd_in_T_offset : Inport  Port=2  PortName=cmd_in  Element=T_offset
  AddOfs : Sum
  WindingLag : DiscreteTransferFcn  Numerator=[1-P.drive.esc.a_Ts]  Denominator=[1 -P.drive.esc.a_Ts]  InitialStates=P.drive.thermal.T_amb0/(1-P.drive.esc.a_Ts)  SampleTime=P.drive.Ts_esc
  T_mot_meas : Outport
  wires:
  T_w/1 -> WindingLag/1  "T_w"
  WindingLag/1 -> AddOfs/1  "WindingLag"
  cmd_in_T_offset/1 -> AddOfs/2  "T_offset"
  AddOfs/1 -> T_mot_meas/1  "T_mot_meas"

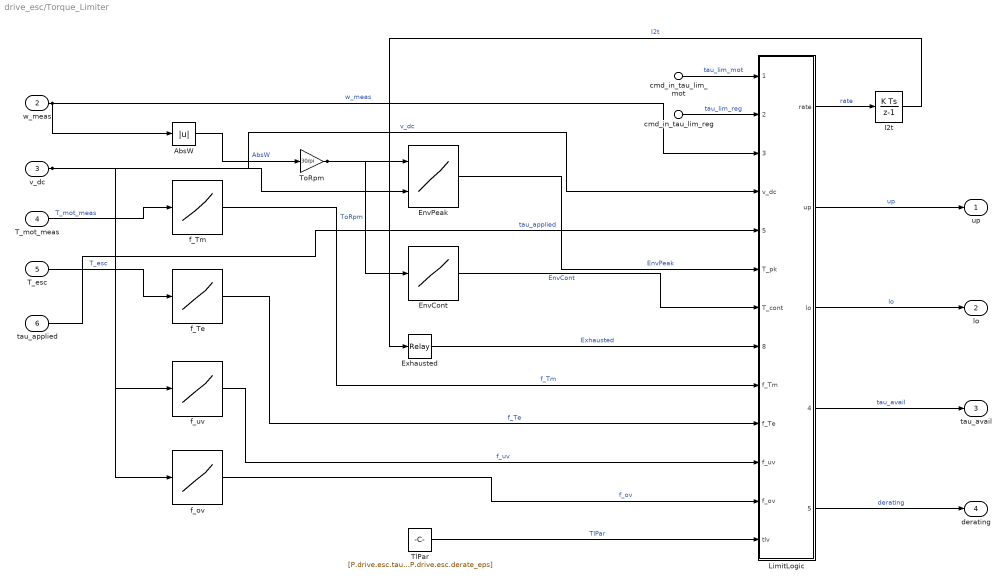
== system drive_esc/Torque_Limiter ==
  cmd_in_tau_lim_mot : Inport  PortName=cmd_in  Element=tau_lim_mot
  cmd_in_tau_lim_reg : Inport  PortName=cmd_in  Element=tau_lim_reg
  w_meas : Inport  Port=2
  v_dc : Inport  Port=3
  T_mot_meas : Inport  Port=4
  T_esc : Inport  Port=5
  tau_applied : Inport  Port=6
  AbsW : Abs  SaturateOnIntegerOverflow=off
  EnvCont : Lookup_n-D  NumberOfTableDimensions=1  BreakpointsForDimension1=P.drive.motor.w_t_rpm  Table=P.drive.motor.T_cont_nom  ExtrapMethod=Clip  InternalRulePriority=Speed  RndMeth=Simplest
  EnvPeak : Lookup_n-D  BreakpointsForDimension1=P.drive.motor.w_t_rpm  BreakpointsForDimension2=P.drive.motor.vdc_t  Table=P.drive.motor.T_pk_2D  ExtrapMethod=Clip  InternalRulePriority=Speed  RndMeth=Simplest
      settings: InputPortMap=u0,u1
  Exhausted : Relay  OnSwitchValue=P.drive.esc.x_on  OffSwitchValue=P.drive.esc.x_off  SampleTime=P.drive.Ts_esc
  I2t : DiscreteIntegrator  gainval=1  SampleTime=P.drive.Ts_esc  LimitOutput=on  UpperSaturationLimit=1  LowerSaturationLimit=0  ICPrevOutput=DiscIntNeverNeededParam  ICPrevScaledInput=DiscIntNeverNeededParam
  LimitLogic : MATLAB Function  TreatAsAtomicUnit=on
  TlPar : Constant  Value=[P.drive.esc.tau_cont_min, 1/P.drive.esc.k_boost, 1/P.drive.esc.t_recover, P.drive.esc.w_min_dc, P.drive.esc.I_dc_max_mot, P.drive.esc.I_dc_max_regen, P.drive.esc.w_quad, 1 - P.drive.esc.derate_eps]  OutDataTypeStr=double
  ToRpm : Gain  Gain=30/pi
  f_Te : Lookup_n-D  NumberOfTableDimensions=1  BreakpointsForDimension1=P.drive.esc.T_esc_derate  Table=[1 0]  ExtrapMethod=Clip  InternalRulePriority=Speed  RndMeth=Simplest
  f_Tm : Lookup_n-D  NumberOfTableDimensions=1  BreakpointsForDimension1=P.drive.esc.T_mot_derate  Table=[1 0]  ExtrapMethod=Clip  InternalRulePriority=Speed  RndMeth=Simplest
  f_ov : Lookup_n-D  NumberOfTableDimensions=1  BreakpointsForDimension1=P.drive.esc.V_ov_derate  Table=[1 0]  ExtrapMethod=Clip  InternalRulePriority=Speed  RndMeth=Simplest
  f_uv : Lookup_n-D  NumberOfTableDimensions=1  BreakpointsForDimension1=P.drive.esc.V_uv_derate  Table=[0 1]  ExtrapMethod=Clip  InternalRulePriority=Speed  RndMeth=Simplest
  up : Outport
  lo : Outport  Port=2
  tau_avail : Outport  Port=3
  derating : Outport  Port=4
  wires:
  w_meas/1 -> LimitLogic/3(w_meas), AbsW/1  "w_meas"
  v_dc/1 -> f_ov/1, f_uv/1, EnvPeak/2, LimitLogic/4(v_dc)  "v_dc"
  T_mot_meas/1 -> f_Tm/1  "T_mot_meas"
  T_esc/1 -> f_Te/1  "T_esc"
  tau_applied/1 -> LimitLogic/5(tau_applied)  "tau_applied"
  AbsW/1 -> ToRpm/1  "AbsW"
  f_Tm/1 -> LimitLogic/9(f_Tm)  "f_Tm"
  f_Te/1 -> LimitLogic/10(f_Te)  "f_Te"
  f_uv/1 -> LimitLogic/11(f_uv)  "f_uv"
  f_ov/1 -> LimitLogic/12(f_ov)  "f_ov"
  ToRpm/1 -> EnvCont/1, EnvPeak/1  "ToRpm"
  Exhausted/1 -> LimitLogic/8(exhausted)  "Exhausted"
  TlPar/1 -> LimitLogic/13(tlv)  "TlPar"
  EnvPeak/1 -> LimitLogic/6(T_pk)  "EnvPeak"
  EnvCont/1 -> LimitLogic/7(T_cont)  "EnvCont"
  cmd_in_tau_lim_mot/1 -> LimitLogic/1(tau_lim_mot)  "tau_lim_mot"
  cmd_in_tau_lim_reg/1 -> LimitLogic/2(tau_lim_reg)  "tau_lim_reg"
  LimitLogic/1(rate) -> I2t/1  "rate"
  LimitLogic/2(up) -> up/1  "up"
  LimitLogic/3(lo) -> lo/1  "lo"
  LimitLogic/4(tau_avail) -> tau_avail/1  "tau_avail"
  LimitLogic/5(derating) -> derating/1  "derating"
  I2t/1 -> Exhausted/1  "I2t"

== matlab function drive_esc/ESC_SM/esc_sm_fcn ==
  data: enable input; state output; mode input; w_ref input; tau_ff input; park_req input; reset_edge input; sto_ok input; v_dc input; can_to input; fault_cond input; w_meas input; smv input; torque_en output; brake_rel output; duty output; hold0 output; qs output; use_speed output; fault_word output; brake_released output
function [state, torque_en, brake_rel, duty, hold0, qs, use_speed, fault_word, brake_released] = esc_sm_fcn(enable, mode, w_ref, tau_ff, park_req, reset_edge, sto_ok, v_dc, can_to, fault_cond, w_meas, smv)
%#codegen
[state, torque_en, brake_rel, duty, hold0, qs, use_speed, fault_word, brake_released] = esc_sm(enable, mode, w_ref, tau_ff, park_req, reset_edge, sto_ok, v_dc, can_to, fault_cond, w_meas, smv);

== matlab function drive_esc/Torque_Limiter/LimitLogic ==
  settings: description=Quadrant torque limits, I2t rate and DERATING flag of one ESC: subsystems/drive/esc_torque_limit.m (D70)
  data: tau_lim_mot input; rate output; tau_lim_reg input; w_meas input; v_dc input; tau_applied input; T_pk input; T_cont input; exhausted input; f_Tm input; f_Te input; f_uv input; f_ov input; tlv input; up output; lo output; tau_avail output; derating output
function [rate, up, lo, tau_avail, derating] = esc_torque_limit_fcn(tau_lim_mot, tau_lim_reg, w_meas, v_dc, tau_applied, T_pk, T_cont, exhausted, f_Tm, f_Te, f_uv, f_ov, tlv)
%#codegen
[rate, up, lo, tau_avail, derating] = esc_torque_limit(tau_lim_mot, tau_lim_reg, w_meas, v_dc, tau_applied, T_pk, T_cont, exhausted, f_Tm, f_Te, f_uv, f_ov, tlv);
end

% ---- verbatim copy of subsystems/drive/esc_torque_limit.m (generated by build_drive, do not edit here) ----
function [rate, up, lo, tau_avail, derating] = esc_torque_limit(tau_lim_mot, tau_lim_reg, w_meas, v_dc, ...
    tau_applied, T_pk, T_cont, exhausted, f_Tm, f_Te, f_uv, f_ov, tlv)
%ESC_TORQUE_LIMIT  Quadrant torque limits of one traction ESC (drive_esc/Torque_Limiter, drive spec 2.9).
%
%   [rate, up, lo, tau_avail, derating] = esc_torque_limit(tau_lim_mot, tau_lim_reg, w_meas, v_dc, ...
%                                         tau_applied, T_pk, T_cont, exhausted, f_Tm, f_Te, f_uv, f_ov, tlv)
%     tau_lim_mot, tau_lim_reg   cmd_in: the motoring and regenerative limits commanded by the MCU (N m)
%     w_meas, v_dc, tau_applied  measured speed (rad/s), DC-link voltage (V), applied torque (N m)
%     T_pk       envelope peak torque: the 2-D Lookup Table EnvPeak (|w| in rpm, v_dc)
%     T_cont     continuous rating: the 1-D Lookup Table EnvCont (|w| in rpm)
%     exhausted  boost exhausted, 1 or 0: the Relay Exhausted on the I2t state x
%     f_Tm, f_Te, f_uv, f_ov     derating factors: the 1-D Lookup Tables of T_mot_meas, T_esc and v_dc
%     tlv        constants (Constant block TlPar): [tau_cont_min, 1/k_boost, 1/t_recover, w_min_dc,
%                I_dc_max_mot, I_dc_max_regen, w_quad, 1 - derate_eps] of P.drive.esc
%     rate       dx/dt of the I2t state, into the Discrete-Time Integrator I2t (x in [0, 1]):
%                (r^2 - 1)/k_boost when r > 1, else (r^2 - 1)/t_recover, r = |tau_applied|/max(T_cont, tau_cont_min)
%     up, lo     upper and lower torque limits (N m): w >= w_quad up = tau_mot, lo = -tau_reg; w <= -w_quad
%                up = tau_reg, lo = -tau_mot; in between +-tau_mot, with
%                tau_mot = min(tau_lim_mot, tau_I2t f_Tm f_Te f_uv, I_dc_max_mot v_dc/max(|w|, w_min_dc)),
%                tau_reg = min(tau_lim_reg, tau_I2t f_Tm f_Te f_ov, I_dc_max_regen v_dc/max(|w|, w_min_dc)),
%                tau_I2t = T_cont when exhausted, else T_pk
%     tau_avail  the ESC's own motoring capability, without the commanded tau_lim_mot (N m)
%     derating   boost exhausted or f_Tm f_Te f_uv < 1 - derate_eps (boolean)
%
%   The MATLAB Function LimitLogic of drive_esc/Torque_Limiter calls it every 1 ms (D70). The Lookup Tables, the
%   I2t integrator and its Relay stay blocks around it, and so do Abs and Gain of the speed in rpm in front of
%   the Lookup Tables (computed here, it would close an algebraic loop through them). The integrator (Forward
%   Euler) has no direct feedthrough, so the loop rate -> I2t -> Exhausted -> exhausted is no algebraic loop. It
%   does what the block network did, operation for operation and in the same order
%   (tests/integration/t_mf_equiv, testDriveEscEquivalent): products left to right as the Product blocks, the
%   Gains as multiplications by the same constants, the Saturations as comparisons that pass NaN as the blocks
%   do, MinMax as local_min (measured, R2026b: it skips NaN as MATLAB's min does, but a tie of +0 and -0 gives the
%   later input, where min gives the first). The comments name the former blocks.
%
%   See also esc_feedback, esc_sm, build_drive.

%#codegen
tau_cont_min = tlv(1);
k_up = tlv(2);
k_dn = tlv(3);
w_min_dc = tlv(4);
I_dcm = tlv(5);
I_dcr = tlv(6);
w_quad = tlv(7);
k_derated = tlv(8);
% I2t charge and recovery rate
tau_abs = abs(tau_applied);                              % AbsTau
cont = T_cont;                                           % ContFloor: Saturation [tau_cont_min, inf]
if cont < tau_cont_min
    cont = tau_cont_min;
end
ratio = tau_abs/cont;                                    % Ratio
sq = ratio*ratio;                                        % Square
m1 = sq + -1;                                            % Minus1 (Bias -1)
if m1 > 0                                                % RateSel (u2 > 0)
    rate = m1*k_up;                                      % RateUp (Gain 1/k_boost)
else
    rate = m1*k_dn;                                      % RateDn (Gain 1/t_recover)
end
% thermal and voltage derating of the envelope
if exhausted > 0.5                                       % TauI2t (u2 > 0.5)
    tau_i2t = T_cont;
else
    tau_i2t = T_pk;
end
kT = f_Tm*f_Te;                                          % kT
tau_th_mot = tau_i2t*kT*f_uv;                            % TauThMot
tau_th_reg = tau_i2t*kT*f_ov;                            % TauThReg
% DC-current limits: tau = I_dc_max v_dc/max(|w|, w_min_dc)
w_fl = abs(w_meas);                                      % AbsW
if w_fl < w_min_dc                                       % WFloor: Saturation [w_min_dc, inf]
    w_fl = w_min_dc;
end
tau_dcm = v_dc*I_dcm/w_fl;                               % Idm, TauDcm
tau_dcr = v_dc*I_dcr/w_fl;                               % Idr, TauDcr
tau_mot = local_min(local_min(tau_lim_mot, tau_th_mot), tau_dcm);   % TauMot
tau_reg = local_min(local_min(tau_lim_reg, tau_th_reg), tau_dcr);   % TauReg
% quadrants
if w_meas*-1 >= w_quad                                   % NegW, UpSel (u2 >= w_quad)
    up = tau_reg;
else
    up = tau_mot;
end
if w_meas >= w_quad                                      % LoSel (u2 >= w_quad)
    lo = tau_reg*-1;                                     % NegReg
else
    lo = tau_mot*-1;                                     % NegMot
end
% tau_avail: the ESC's own capability; min(tau_lim_mot, ...) would deadlock with the MCU, which sets
% tau_lim_mot = min(.., tau_avail)
tau_avail = local_min(tau_th_mot, tau_dcm);              % TauAvail
derating = kT*f_uv < k_derated || exhausted > 0.5;       % kAll, Derated, IsExh, DerOr
end

function y = local_min(a, b)
% the MinMax block (min) on two inputs: b, unless a < b or b is NaN; so NaN is skipped and a tie gives b
if a < b || isnan(b)
    y = a;
else
    y = b;
end
end

== matlab function drive_esc/Feedback/FbPack ==
  settings: description=Status word, alive counter and Bus_DriveSideFb of one ESC: subsystems/drive/esc_feedback.m (D70)
  data: mode input; fb output Bus: Bus_DriveSideFb; state input; brake_released input; fault_word input; derating input; lim_active input; sto_ok input; stall_warn input; w_meas input; enc_cnt input; tau_est input; tau_avail input; i_q input; i_dc input; v_dc input; T_mot_meas input; T_esc input; tick input; k_alive input
function fb = esc_feedback_fcn(mode, state, brake_released, fault_word, derating, lim_active, sto_ok, stall_warn, w_meas, enc_cnt, tau_est, tau_avail, i_q, i_dc, v_dc, T_mot_meas, T_esc, tick, k_alive)
%#codegen
fb = esc_feedback(mode, state, brake_released, fault_word, derating, lim_active, sto_ok, stall_warn, w_meas, enc_cnt, tau_est, tau_avail, i_q, i_dc, v_dc, T_mot_meas, T_esc, tick, k_alive);
end

% ---- verbatim copy of subsystems/drive/esc_feedback.m (generated by build_drive, do not edit here) ----
function fb = esc_feedback(mode, state, brake_released, fault_word, derating, lim_active, ~, stall_warn, ...
    w_meas, enc_cnt, tau_est, tau_avail, i_q, i_dc, v_dc, T_mot_meas, T_esc, tick, k_alive)
%ESC_FEEDBACK  Status word, alive counter and feedback bus of one traction ESC (drive_esc/Feedback, spec 2.9).
%
%   fb = esc_feedback(mode, state, brake_released, fault_word, derating, lim_active, sto_ok, stall_warn, ...
%                     w_meas, enc_cnt, tau_est, tau_avail, i_q, i_dc, v_dc, T_mot_meas, T_esc, tick, k_alive)
%     mode            cmd_in.mode: 0 OFF, 1 SPEED, 2 TORQUE (double)
%     state           sm.state: EscState 0 INIT .. 8 STO (uint8)
%     brake_released  sm.brake_released (boolean)
%     fault_word      sm.fault_word (uint16; bit 10 STO_ACTIVE is set by ESC_SM while sto_ok is false)
%     derating        Torque_Limiter: boost exhausted or a derating factor active (boolean)
%     lim_active      Speed_Ctrl: the commanded torque is clipped by the limiter (boolean)
%     sto_ok          (the 7th input, ~) not used: STO_ACTIVE comes from the state and from fault-word bit 10
%                     (the former block network terminated it)
%     stall_warn      Protections: stall warning (boolean)
%     w_meas, tau_est, tau_avail, i_q, i_dc, v_dc, T_mot_meas, T_esc   measured values (double), sent as single
%     enc_cnt         encoder count (int32)
%     tick            the alive tick 0 .. 256*n_alive - 1 (the Counter Limited block Tick, a state, stays a block)
%     k_alive         1/P.drive.esc.n_alive (Constant block FbPar)
%     fb              Bus_DriveSideFb (FB frames, ICD 4)
%
%   Status word (uint16): b0 READY (state 2-6), b1 OP_ENABLED (4), b2 FAULT (7), b3 DERATING, b4 BRAKE_RELEASED,
%   b5 MODE_SPEED, b6 MODE_TORQUE, b7 TORQUE_LIMIT_ACTIVE, b8 STO_ACTIVE (state 8 or fault-word bit 10),
%   b9 QUICKSTOP (6), b10 STALL_WARNING. Alive counter: floor(tick/n_alive), +1 per 10 ms (one FB frame).
%
%   The MATLAB Function FbPack of drive_esc/Feedback calls it every 1 ms (D70). It does what the block network
%   did, operation for operation (tests/integration/t_mf_equiv, testDriveEscEquivalent): each cast is that of its
%   Data Type Conversion, Nearest and saturating. MATLAB's casts round to nearest with ties away from zero and
%   saturate, which is the same for the unsigned targets uint16 and uint8 (a negative tie saturates to 0 either
%   way); a float to single cast rounds as the block does. The comments name the former blocks.
%
%   See also esc_torque_limit, esc_sm, build_drive.

%#codegen
st = double(state);                                      % StateD
ready = st >= 2 && st <= 6;                              % Ready1, Ready2, IsReady
op = st == 4;                                            % IsOp
fault = st == 7;                                         % IsFault
sto = st == 8;                                           % IsSto
quick = st == 6;                                         % IsQs
speed = mode == 1;                                       % IsSpeed
torque = mode == 2;                                      % IsTorque
sto_act = sto || bitand(fault_word, uint16(1024)) ~= 0;  % StoBit ([10 10]), StoBitOn, StoAct
b = [uint16(ready), uint16(op), uint16(fault), uint16(derating), uint16(brake_released), uint16(speed), ...
    uint16(torque), uint16(lim_active), uint16(sto_act), uint16(quick), uint16(stall_warn)];   % sb0 .. sb10
status = uint16(0);                                      % StatusMux, StatusShift (0:10 left), Status (OR)
for k = 1:11
    status = bitor(status, bitshift(b(k), k - 1));
end
alive = uint8(floor(double(tick)*k_alive));              % TickD, PerFrame, Floor, alive
fb = struct('state', state, 'status', status, 'fault_code', fault_word, 'w_m', single(w_meas), ...
    'enc_cnt', enc_cnt, 'tau_est', single(tau_est), 'tau_avail', single(tau_avail), 'i_q', single(i_q), ...
    'i_dc', single(i_dc), 'v_dc', single(v_dc), 'T_motor', single(T_mot_meas), 'T_esc', single(T_esc), ...
    'brake_released', brake_released, 'alive', alive, 'rx_ok', true);    % the *_s conversions, RxOk, Fb
end
